simulink model "GearShift_Stateflow"  (R2025b)
settings: Solver=FixedStepAuto  StartTime=0.0  StopTime=inf  FixedStep=0.01  RelTol=1e-3
settings Model: Creator=XC_Serendipity  LastModifiedBy=XC_Serendipity
settings OptimizationCC: DefaultParameterBehavior=Inlined  EnhancedBackFolding=on  PassReuseOutputArgsAs=Individual arguments  ZeroExternalMemoryAtStartup=off  ZeroInternalMemoryAtStartup=off  OptimizeBlockOrder=speed  DifferentSizesBufferReuse=on  OptimizationCustomize=off  EfficientTunableParamExpr=on
settings DebuggingCC: ParameterTunabilityLossMsg=error
settings HardwareCC: ProdBitPerPointer=32.0  ProdBitPerSizeT=32.0  ProdBitPerPtrDiffT=32.0  ProdLargestAtomicInteger=Long  ProdLargestAtomicFloat=Double  ProdWordSize=32.0  ProdLongLongMode=on  ProdHWDeviceType=NXP->Cortex-M4
settings SFSimCC: MATLABDynamicMemAlloc=off
settings RTWCC: SystemTargetFile=ert.tlc  GenCodeOnly=on  TemplateMakefile=ert_default_tmf  Description=Embedded Coder
settings CodeAppCC: ForceParamTrailComments=on  IgnoreCustomStorageClasses=off  OperatorAnnotations=on  SimulinkDataObjDesc=on  SFDataObjDesc=on  InsertBlockDesc=on
settings ERTTargetCC: ERTCustomFileTemplate=example_file_process.tlc  TargetLangStandard=C99 (ISO)  GenerateSampleERTMain=on

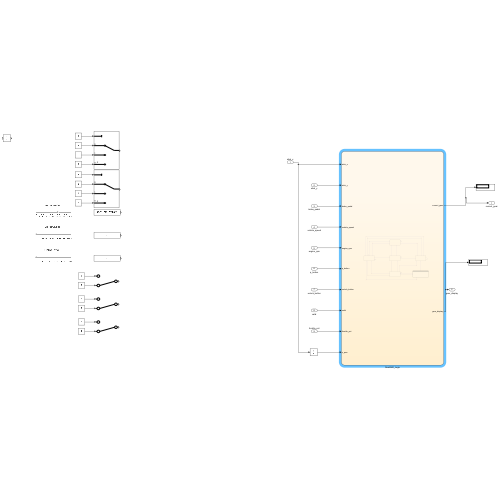
[thumbnail: Simulink's stored preview of the top-level diagram]
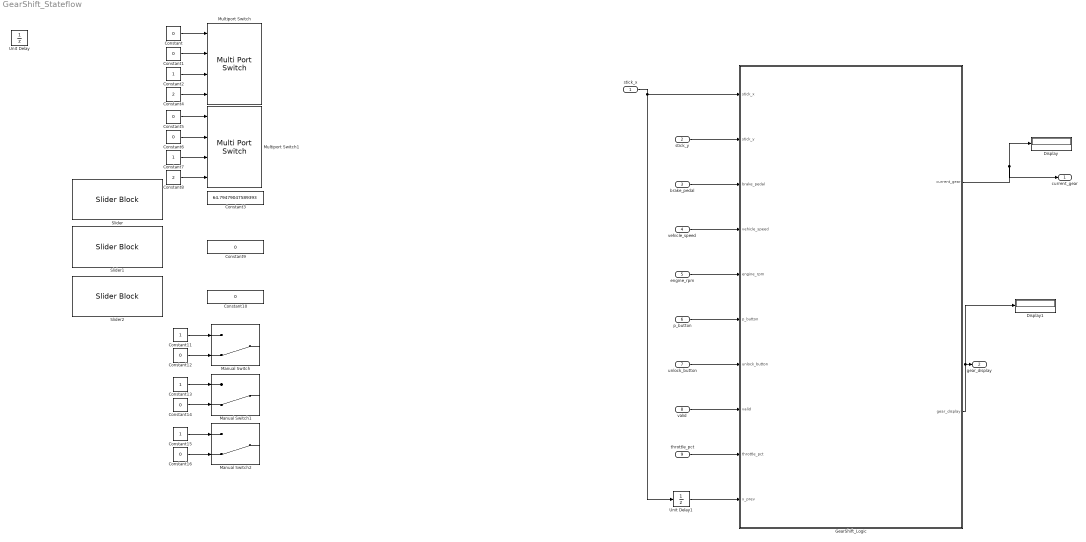
== system GearShift_Stateflow ==
  stick_x : Inport  OutDataTypeStr=uint8
  stick_y : Inport  Port=2  OutDataTypeStr=uint8
  brake_pedal : Inport  Port=3  OutDataTypeStr=uint16
  vehicle_speed : Inport  Port=4  OutDataTypeStr=uint16
  engine_rpm : Inport  Port=5  OutDataTypeStr=uint16
  p_button : Inport  Port=6  OutDataTypeStr=boolean
  unlock_button : Inport  Port=7  OutDataTypeStr=boolean
  valid : Inport  Port=8  OutDataTypeStr=boolean
  throttle_pct : Inport  Port=9  OutDataTypeStr=uint8
  Constant{,1,5..6} (4 alike) : Constant  Value=0
  Constant10 : Constant  Value=0  OutDataTypeStr=uint16
  Constant11 : Constant  OutDataTypeStr=boolean
  Constant12 : Constant  Value=0  OutDataTypeStr=boolean
  Constant13 : Constant  OutDataTypeStr=boolean
  Constant14 : Constant  Value=0  OutDataTypeStr=boolean
  Constant15 : Constant  OutDataTypeStr=boolean
  Constant16 : Constant  Value=0  OutDataTypeStr=boolean
  Constant2 : Constant
  Constant3 : Constant  Value=64.79479047589393  OutDataTypeStr=uint16
  Constant4 : Constant  Value=2
  Constant7 : Constant
  Constant8 : Constant  Value=2
  Constant9 : Constant  Value=0  OutDataTypeStr=uint16
  Display : Display
  Display1 : Display
  GearShift_Logic : Stateflow chart  TreatAsAtomicUnit=on
  Manual Switch : ManualSwitch  CurrentSetting=0
  Manual Switch1 : ManualSwitch  CurrentSetting=0
  Manual Switch2 : ManualSwitch  CurrentSetting=0
  Multiport Switch : MultiPortSwitch  DataPortOrder=Zero-based contiguous  zeroidx=on  OutDataTypeStr=uint8  SaturateOnIntegerOverflow=off  InputSameDT=off
  Multiport Switch1 : MultiPortSwitch  DataPortOrder=Zero-based contiguous  zeroidx=on  OutDataTypeStr=uint8  SaturateOnIntegerOverflow=off  InputSameDT=off
  Slider : SliderBlock
  Slider1 : SliderBlock  ScaleMax=120
  Slider2 : SliderBlock  ScaleMax=8000
  Unit Delay : UnitDelay  SampleTime=-1  HasFrameUpgradeWarning=on
  Unit Delay1 : UnitDelay  SampleTime=-1  HasFrameUpgradeWarning=on
  current_gear : Outport  OutDataTypeStr=uint8
  gear_display : Outport  Port=2  OutDataTypeStr=uint8
  wires:
  GearShift_Logic/1(current_gear) -> Display/1, current_gear/1
  GearShift_Logic/2(gear_display) -> Display1/1, gear_display/1
  Constant/1 -> Multiport Switch/1
  Constant1/1 -> Multiport Switch/2
  Constant2/1 -> Multiport Switch/3
  Constant4/1 -> Multiport Switch/4
  Constant5/1 -> Multiport Switch1/1
  Constant8/1 -> Multiport Switch1/4
  Constant6/1 -> Multiport Switch1/2
  Constant7/1 -> Multiport Switch1/3
  Constant11/1 -> Manual Switch/1
  Constant12/1 -> Manual Switch/2
  Constant14/1 -> Manual Switch1/2
  Constant13/1 -> Manual Switch1/1
  Constant15/1 -> Manual Switch2/1
  Constant16/1 -> Manual Switch2/2
  stick_x/1 -> Unit Delay1/1, GearShift_Logic/1(stick_x)
  stick_y/1 -> GearShift_Logic/2(stick_y)
  brake_pedal/1 -> GearShift_Logic/3(brake_pedal)
  vehicle_speed/1 -> GearShift_Logic/4(vehicle_speed)
  engine_rpm/1 -> GearShift_Logic/5(engine_rpm)
  p_button/1 -> GearShift_Logic/6(p_button)
  unlock_button/1 -> GearShift_Logic/7(unlock_button)
  valid/1 -> GearShift_Logic/8(valid)
  Unit Delay1/1 -> GearShift_Logic/10(x_prev)
  throttle_pct/1 -> GearShift_Logic/9(throttle_pct)

== stateflow chart GearShift_Stateflow/GearShift_Logic ==
  state R
    entry: current_gear = 1; gear_display = 1;
    during: comm_timeout_timer++;
  state P
    entry: current_gear = 0; gear_display = 0;
    during: comm_timeout_timer++;
  state N
    entry: current_gear = 2; gear_display = 2;
    during: comm_timeout_timer++;
  state FAULT
    entry: current_gear = 255; gear_display = 255;
    during: comm_timeout_timer++;
  state M
    state M1
      entry: current_gear = 11; gear_display = 11;
      during: comm_timeout_timer++;
    state M2
      entry: current_gear = 12; gear_display = 12;
      during: comm_timeout_timer++;
    state M3
      entry: current_gear = 13; gear_display = 13;
      during: comm_timeout_timer++;
    state Init
    state M6
      entry: current_gear = 16; gear_display = 16;
      during: comm_timeout_timer++;
    state M5
      entry: current_gear = 15; gear_display = 15;
      during: comm_timeout_timer++;
    state M4
      entry: current_gear = 14; gear_display = 14;
      during: comm_timeout_timer++;
    M1 -> M2 [order 2] : [stick_x==2 && x_prev==0 && engine_rpm>=2000 && vehicle_speed>=25]
    M2 -> M3 [order 3] : [stick_x==2 && x_prev==0 && engine_rpm>=2000 && vehicle_speed>=50
        | ]
    M1 -> M1 [order 3] : [valid]{comm_timeout_timer = 0;}
    M2 -> M2 [order 5] : [valid]{comm_timeout_timer = 0;}
    M3 -> M3 [order 5] : [valid]{comm_timeout_timer = 0;}
    M3 -> M2 [order 4] : [stick_x==1 && x_prev==0 && vehicle_speed<=40]
    M2 -> M1 [order 4] : [stick_x==1 && x_prev==0 && vehicle_speed<=15]
    M1 -> M2 [order 1] : [engine_rpm > 6500]
    M2 -> M3 [order 1] : [engine_rpm > 6500]
    M2 -> M1 [order 2] : [engine_rpm < 1200]
    M3 -> M2 [order 2] : [engine_rpm < 1200]
    Init -> M2 [order 2] : [vehicle_speed >= 10 && vehicle_speed < 30]
    (junction 226) -> M1 : [vehicle_speed < 10]
    (junction 238) -> M3 : [vehicle_speed >= 30 && vehicle_speed < 50]
    M4 -> M3 [order 2] : [engine_rpm < 1200]
    M3 -> M4 [order 1] : [engine_rpm > 6500]
    M3 -> M4 [order 3] : [stick_x==2 && x_prev==0 && engine_rpm>=2000 && vehicle_speed>=80]
    M4 -> M3 [order 4] : [stick_x==1 && x_prev==0 && vehicle_speed<=70]
    Init -> (junction 226) [order 1]
    Init -> (junction 238) [order 3]
    (default) -> Init
    Init -> (junction 242) [order 4]
    (junction 242) -> M4 : [vehicle_speed >= 50 && vehicle_speed < 70]
    Init -> (junction 234) [order 6]
    (junction 234) -> M6 : [vehicle_speed >= 90]
    Init -> M5 [order 5] : [vehicle_speed >= 70 && vehicle_speed < 90]
    M4 -> M5 [order 3] : [stick_x==2 && x_prev==0 && engine_rpm>=2000 && vehicle_speed>=120]
    M5 -> M6 [order 3] : [stick_x==2 && x_prev==0 && engine_rpm>=2000 && vehicle_speed>=160]
    M4 -> M4 [order 5] : [valid]{comm_timeout_timer = 0;}
    M6 -> M6 [order 3] : [valid]{comm_timeout_timer = 0;}
    M5 -> M5 [order 5] : [valid]{comm_timeout_timer = 0;}
    M6 -> M5 [order 2] : [stick_x==1 && x_prev==0 && vehicle_speed<=140]
    M5 -> M4 [order 4] : [stick_x==1 && x_prev==0 && vehicle_speed<=100]
    M5 -> M6 [order 1] : [engine_rpm > 6500]
    M4 -> M5 [order 1] : [engine_rpm > 6500]
    M6 -> M5 [order 1] : [engine_rpm < 1200]
    M5 -> M4 [order 2] : [engine_rpm < 1200]
  state D
    entry: current_gear = 3; gear_display = 3;
    during: comm_timeout_timer++;
  (junction 196) -> (junction 198)
  (junction 198) -> P : [p_button && vehicle_speed<5 && x_prev==0&& brake_pedal > 30]
  FAULT -> (junction 196) [order 1]
  (junction 154) -> (junction 158)
  P -> (junction 154) [order 1]
  (junction 158) -> FAULT : [comm_timeout_timer>200]
  R -> R [order 4] : [valid]{comm_timeout_timer = 0;}
  (junction 178) -> R : [stick_x==2 && brake_pedal>30 && vehicle_speed<5 && unlock_button && x_prev==0]
  P -> (junction 178) [order 3]
  R -> (junction 184) [order 2]
  R -> (junction 203) [order 1]
  (junction 184) -> P : [p_button && vehicle_speed<5 && x_prev==0&& brake_pedal > 30]
  (junction 203) -> FAULT : [comm_timeout_timer>200]
  R -> N [order 3] : [stick_x==1 && vehicle_speed<5 && x_prev==0]
  N -> R [order 4] : [stick_x==2 && vehicle_speed<5 && x_prev==0]
  (default) -> P
  N -> N [order 5] : [valid]{comm_timeout_timer = 0;}
  N -> P [order 2] : [p_button && vehicle_speed<5 && x_prev==0&& brake_pedal > 30]
  FAULT -> FAULT [order 2] : [valid]{comm_timeout_timer = 0;}
  N -> FAULT [order 1] : [comm_timeout_timer>200]
  P -> P [order 4] : [valid]{comm_timeout_timer = 0;}
  (junction 190) -> P : [p_button && vehicle_speed<5 && x_prev==0&& brake_pedal > 30&& (throttle_pct == 0) && (vehicle_speed == 0)]
  P -> (junction 168) [order 2]
  (junction 173) -> P : [p_button && vehicle_speed<5 && x_prev==0&& brake_pedal > 30&& (throttle_pct == 0) && (vehicle_speed == 0)]
  N -> D [order 3] : [stick_x==1 && x_prev==0]
  D -> N [order 3] : [stick_x==2 && x_prev==0]
  (junction 163) -> FAULT : [comm_timeout_timer>200]
  M -> FAULT [order 1] : [comm_timeout_timer>200]
  (junction 161) -> (junction 163)
  D -> (junction 161) [order 1]
  D -> D [order 5] : [valid]{comm_timeout_timer = 0;}
  D -> (junction 173) [order 2]
  M -> D [order 3] : [stick_y==1]
  D -> M [order 4] : [stick_y==2 && x_prev==0]
  (junction 168) -> D : [stick_x==1 && brake_pedal>30 && vehicle_speed<5 && unlock_button && x_prev==0]
  M -> (junction 188) [order 2]
  (junction 188) -> (junction 190)
  data: stick_x input uint8; stick_y input uint8; brake_pedal input uint16; vehicle_speed input uint16; engine_rpm input uint16; p_button input boolean; unlock_button input boolean; valid input boolean; throttle_pct input uint8; current_gear output uint8; gear_display output uint8; comm_timeout_timer local uint16 size=1 =1; x_prev input uint8
  data stick_x settings: description=摇杆 X 轴：0回中/1后拉/2前推
  data stick_y settings: description=摇杆 Y 轴：0回中/1左推/2右推
  data brake_pedal settings: description=刹车深度 0~100
  data vehicle_speed settings: description=车速 km/h
  data engine_rpm settings: description=发动机转速
  data p_button settings: description=P 键
  data unlock_button settings: description=解锁键
  data valid settings: description=通信有效标志
  data current_gear settings: description=当前挡位编码
  data gear_display settings: description=显示挡位编码
  data comm_timeout_timer settings: description=通信超时计数器
